simulink model "Task4_Simscape_model"  (R2026a)
settings: Solver=FixedStepAuto  StopTime=8  FixedStep=0.001
model workspace (MATLAB code in the model file):
  | clear; clc; close all;
values from neighbouring files (symbols this model uses):
  A0 = 0.310447780017169    (= 0.310447780017)    [Parameters.m]    (also in Parameters_optimization.m)
  B10 = -0.192075602039053    (= -0.192075602039)    [Parameters.m]    (also in Parameters_optimization.m)
  B20 = -0.011912003704451    (= -0.0119120037045)    [Parameters.m]    (also in Parameters_optimization.m)
  black = partTemplate    [Parameters.m]    (also in Parameters_optimization.m = struct)
  blueBlock = partTemplate    [Parameters.m]    (also in Parameters_optimization.m = struct)
  cyan = partTemplate    [Parameters.m]    (also in Parameters_optimization.m = struct)
  g = 9.81    [Parameters.m]    (also in Parameters_optimization.m)
  G0 = -1.061422531644424    (= -1.06142253164)    [Parameters.m]    (also in Parameters_optimization.m)
  greenBeam = partTemplate    [Parameters.m]    (also in Parameters_optimization.m = struct)
  greenBlock = partTemplate    [Parameters.m]    (also in Parameters_optimization.m = struct)
  grey = partTemplate    [Parameters.m]    (also in Parameters_optimization.m = struct)
  H0 = -0.357470264672538    (= -0.357470264673)    [Parameters.m]    (also in Parameters_optimization.m)
  I0 = -1.033155420835947    (= -1.03315542084)    [Parameters.m]    (also in Parameters_optimization.m)
  JM = 0.002    [Parameters.m]    (also in Parameters_optimization.m)
  LB1 = 0.8    [Parameters.m]    (also in Parameters_optimization.m)
  LB2 = 0.3    [Parameters.m]    (also in Parameters_optimization.m)
  LB3 = 0.24    [Parameters.m]    (also in Parameters_optimization.m)
  Lblack1 = 0.2    [Parameters.m]    (also in Parameters_optimization.m)
  LC1 = 0.4    [Parameters.m]    (also in Parameters_optimization.m)
  LC2 = 0.225    [Parameters.m]    (also in Parameters_optimization.m)
  LG1 = 0.3    [Parameters.m]    (also in Parameters_optimization.m)
  LG2 = 0.8    [Parameters.m]    (also in Parameters_optimization.m)
  Lgrey1 = 1.175    [Parameters.m]    (also in Parameters_optimization.m)
  lightBlue = partTemplate    [Parameters.m]    (also in Parameters_optimization.m = struct)
  LLB1 = 0.248    [Parameters.m]    (also in Parameters_optimization.m)
  LLB2 = 0.235    [Parameters.m]    (also in Parameters_optimization.m)
  LR1 = 1.05    [Parameters.m]    (also in Parameters_optimization.m)
  LW1 = 1.05    [Parameters.m]    (also in Parameters_optimization.m)
  nA = 200    [Parameters.m]    (also in Parameters_optimization.m = 100)
  nB1 = 200    [Parameters.m]    (also in Parameters_optimization.m = 100)
  nB2 = 200    [Parameters.m]    (also in Parameters_optimization.m)
  nG = 20    [Parameters.m]    (also in Parameters_optimization.m)
  nH = 100    [Parameters.m]    (also in Parameters_optimization.m = 50)
  nI = 20    [Parameters.m]    (also in Parameters_optimization.m)
  red = partTemplate    [Parameters.m]    (also in Parameters_optimization.m = struct)
  trajCoeff = coeff    [Parameters.m]    (also in Parameters_optimization.m = [2000 500 1600; Path_Planning_Robot.m)
  trajTime = t    [Parameters.m]    (also in Parameters_optimization.m = [0 2 4 6 8]; Path_Planning_Robot.m)
  w = 0.1    [Parameters.m]    (also in Parameters_optimization.m)
  white = partTemplate    [Parameters.m]    (also in Parameters_optimization.m = struct)
undefined symbols (not defined in the file or in its folder): X, Y, Z
libraries: sm_lib x152, nesl_utility x69, simulink x1
(part 1 of 5)
settings Model: Creator=Bruker  LastModifiedBy=Bruker
settings ExplorerConfigSet: InternalSimMechanicsExplorerSettings=|
  | <ExplorerConfiguration>
  | 
  |   <canonicalview>default</canonicalview>
  | 
  |   <TilePanel>
  |     <TileInfo>
  |       <Tiles Columns="1" Count="1" Height="610" Rows="1" Width="1078">
  |         <Row Weight="1"/>
  |         <Column Weight="1"/>
  |         <Tile Height="1" Width="1" X="0" Y="0"/>
  |       </Tiles>
  |     </TileInfo>
  |     <SceneInfo>
  |       <SceneViewer>
  |         <IsThisViewStd>
  |           <IsStandardView>off</IsStandardView>
  |           <StandardViewName>Front</StandardViewName>
  |         </IsThisViewStd>
  |         <BGColor>
  |           <R>1</R>
  |           <G>1</G>
  |           <B>1</B>
  |           <A>1</A>
  |         </BGColor>
  |         <Camera>
  |           <DoPerspective>off</DoPerspective>
  |           <Position>
  |             <X>0.050962097420724523</X>
  |             <Y>-3.1475704894834529</Y>
  |             <Z>0.37490286963399816</Z>
  |           </Position>
  |           <Center>
  |             <X>0.050962097420724523</X>
  |             <Y>0</Y>
  |             <Z>0.37490286963399816</Z>
  |           </Center>
  |           <Up>
  |             <X>0</X>
  |             <Y>0</Y>
  |             <Z>1</Z>
  |           </Up>
  |           <XLim>0.57510337083613783</XLim>
  |           <YLim>0.57510337083613783</YLim>
  |           <ViewLimDist>0.01</ViewLimDist>
  |         </Camera>
  |       </SceneViewer>
  |     </SceneInfo>
  |   </TilePanel>
  | 
  |   <MechEditorPanel>
  |     <GfxPanelCameraMap/>
  |     <Cameras/>
  |     <VideoCreator>
  |       <IncludeTiles>All</IncludeTiles>
  |       <IncludeTime>on</IncludeTime>
  |       <IncludeWorldFrame>off</IncludeWorldFrame>
  |       <PlaybackSpeedRatio>1</PlaybackSpeedRatio>
  |       <FrameRate>30</FrameRate>
  |       <FrameSize>auto</FrameSize>
  |       <VideoFormat>UncompressedAVI</VideoFormat>
  |     </VideoCreator>
  |   </MechEditorPanel>
  | 
  |   <PlaybackSettings>
  |     <PlaybackSpeedFactor>1</PlaybackSpeedFactor>
  |   </PlaybackSettings>
  | 
  | </ExplorerConfiguration>

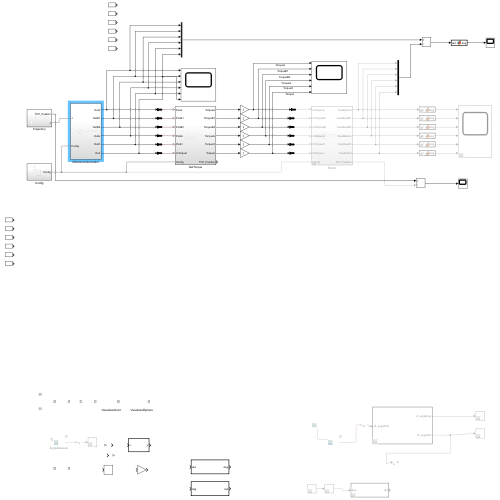
[thumbnail: Simulink's stored preview of the top-level diagram]
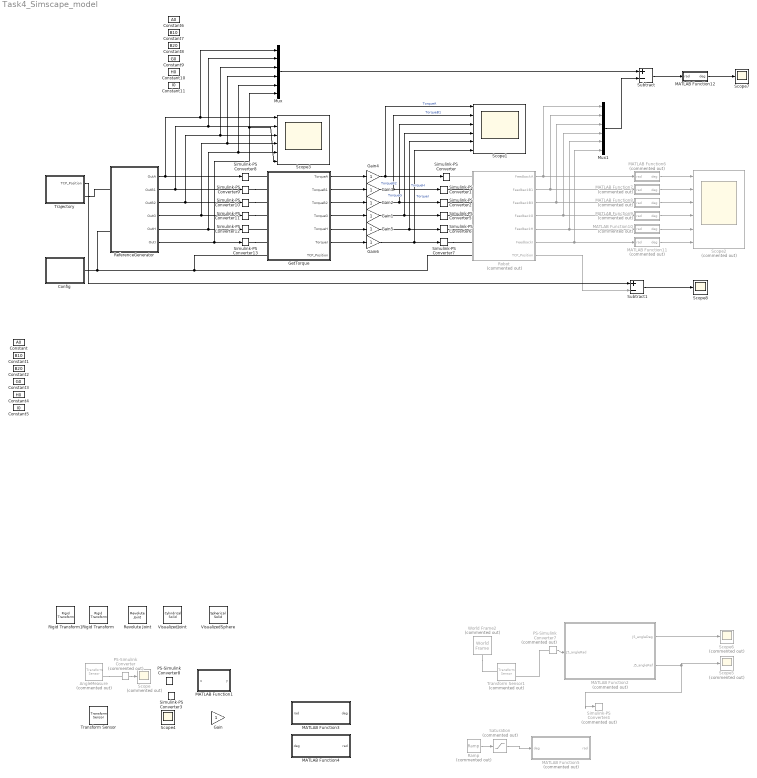
== system Task4_Simscape_model ==
  AngleMeasure : sm_lib/Frames and Transforms/Transform Sensor  Commented=on  MeasurementFrame=World  RotationSequence=XYX  SenseAngle=on  SenseAxis=off  SenseQ=off  SenseR=off  SenseRotationSequence=off  SenseOmegaX=off  SenseOmegaY=off  SenseOmegaZ=off  SenseOmega=off  SenseQDot=off  SenseRDot=off  SenseRotationSequenceDot=off  SenseAlphaX=off  SenseAlphaY=off  SenseAlphaZ=off  SenseAlpha=off  SenseQDDot=off  SenseRDDot=off  SenseX=off  SenseY=off  SenseZ=off  SenseXYZ=off  SenseRad=off  SenseAzim=off  SenseDist=off  SenseInc=off  SenseXDot=off  SenseYDot=off  SenseZDot=off  SenseXYZDot=off  SenseRadDot=off  SenseAzimDot=off  SenseDistDot=off  SenseIncDot=off  SenseXDDot=off  SenseYDDot=off  SenseZDDot=off  SenseXYZDDot=off  SenseRadDDot=off  SenseAzimDDot=off  SenseDistDDot=off  SenseIncDDot=off
  Config : Subsystem
  Constant : Constant  Value=A0
  Constant1 : Constant  Value=B10
  Constant10 : Constant  Value=H0
  Constant11 : Constant  Value=I0
  Constant2 : Constant  Value=B20
  Constant3 : Constant  Value=G0
  Constant4 : Constant  Value=H0
  Constant5 : Constant  Value=I0
  Constant6 : Constant  Value=A0
  Constant7 : Constant  Value=B10
  Constant8 : Constant  Value=B20
  Constant9 : Constant  Value=G0
  Gain{,1..6} (7 alike) : Gain
  GetTorque : Subsystem
  MATLAB Function1 : MATLAB Function  TreatAsAtomicUnit=on
  MATLAB Function10 : MATLAB Function  Commented=on  TreatAsAtomicUnit=on
  MATLAB Function11 : MATLAB Function  Commented=on  TreatAsAtomicUnit=on
  MATLAB Function12 : MATLAB Function  TreatAsAtomicUnit=on
  MATLAB Function2 : MATLAB Function  Commented=on  TreatAsAtomicUnit=on
  MATLAB Function3 : MATLAB Function  TreatAsAtomicUnit=on
  MATLAB Function4 : MATLAB Function  TreatAsAtomicUnit=on
  MATLAB Function5 : MATLAB Function  Commented=on  TreatAsAtomicUnit=on
  MATLAB Function6 : MATLAB Function  Commented=on  TreatAsAtomicUnit=on
  MATLAB Function7 : MATLAB Function  Commented=on  TreatAsAtomicUnit=on
  MATLAB Function8 : MATLAB Function  Commented=on  TreatAsAtomicUnit=on
  MATLAB Function9 : MATLAB Function  Commented=on  TreatAsAtomicUnit=on
  Mux : Mux  Inputs=6
  Mux1 : Mux  Inputs=6
  PS-Simulink Converter : nesl_utility/PS-Simulink Converter  Commented=on  PhysicalDomain=network_engine_domain  SubClassName=ps_output  LeftPortType=input  RightPortType=output  PseudoPeriodic=off  Frequencies=[]  VectorFormat=inherit  Unit=inherit  AffineConversion=off
  PS-Simulink Converter7 : nesl_utility/PS-Simulink Converter  Commented=on  PhysicalDomain=network_engine_domain  SubClassName=ps_output  LeftPortType=input  RightPortType=output  PseudoPeriodic=off  Frequencies=[]  VectorFormat=inherit  Unit=inherit  AffineConversion=off
  PS-Simulink Converter8 : nesl_utility/PS-Simulink Converter  PhysicalDomain=network_engine_domain  SubClassName=ps_output  LeftPortType=input  RightPortType=output  PseudoPeriodic=off  Frequencies=[]  VectorFormat=inherit  Unit=inherit  AffineConversion=off
  Ramp : simulink/Sources/Ramp  Commented=on  slope=1000/8  start=0  InitialOutput=0
  ReferenceGenerator : Subsystem
  Revolute Joint : sm_lib/Joints/Revolute Joint  JointMode=Normal  CompositeWrenchDir=FollowerOnBase  CompositeWrenchFrame=BaseFrame  SenseConstraintForce=off  SenseConstraintTorque=off  SenseTotalForce=off  SenseTotalTorque=off  PositionTargetSpecify=off  PositionTargetPriority=High  PositionTargetValue=0  PositionTargetValueUnits=deg  VelocityTargetSpecify=off  VelocityTargetPriority=High  VelocityTargetValue=0  VelocityTargetValueUnits=deg/s  EquilibriumPosition=0  EquilibriumPositionUnits=deg  SpringStiffness=0  SpringStiffnessUnits=N*m/deg  DampingCoefficient=0  DampingCoefficientUnits=N*m/(deg/s)  LowerLimitSpecify=off  LowerLimitBound=-90  LowerLimitBoundUnits=deg  LowerLimitStiffness=1e4  LowerLimitStiffnessUnits=N*m/deg  LowerLimitDamping=10  LowerLimitDampingUnits=N*m/(deg/s)  LowerLimitTransitionRegionWidth=0.1  LowerLimitTransitionRegionWidthUnits=deg  UpperLimitSpecify=off  UpperLimitBound=90  UpperLimitBoundUnits=deg  UpperLimitStiffness=1e4  UpperLimitStiffnessUnits=N*m/deg  UpperLimitDamping=10  UpperLimitDampingUnits=N*m/(deg/s)  UpperLimitTransitionRegionWidth=0.1  UpperLimitTransitionRegionWidthUnits=deg  TorqueActuationMode=NoTorque  MotionActuationMode=ComputedMotion  SensePosition=off  SenseVelocity=off  SenseAcceleration=off  SenseTorqueForce=off  SenseLowerLimitTorqueForce=off  SenseUpperLimitTorqueForce=off
  Rigid Transform : sm_lib/Frames and Transforms/Rigid Transform  RotationMethod=None  FollAlignAxisA=+X  BaseAlignAxisA=+Y  FollAlignAxisB=+Y  BaseAlignAxisB=+Z  RotationStandardAxis=+Z  RotationAngle=0  RotationAngleUnits=deg  RotationArbitraryAxis=[0 0 1]  RotationSequenceAxes=FollowerAxes  RotationSequence=XYX  RotationSequenceAngles=[0 0 0]  RotationSequenceAnglesUnits=deg  RotationMatrix=[1 0 0;0 1 0;0 0 1]  Quaternion=[1 0 0 0]  TranslationMethod=None  TranslationCartesianOffset=[0 0 0]  TranslationCartesianOffsetUnits=m  TranslationStandardAxis=+Z  TranslationStandardOffset=0  TranslationStandardOffsetUnits=m  TranslationROffset=0  TranslationROffsetUnits=m  TranslationThetaOffset=0  TranslationThetaOffsetUnits=deg  TranslationZOffset=0  TranslationZOffsetUnits=m
  Rigid Transform1 : sm_lib/Frames and Transforms/Rigid Transform  RotationMethod=None  FollAlignAxisA=+X  BaseAlignAxisA=+Y  FollAlignAxisB=+Y  BaseAlignAxisB=+Z  RotationStandardAxis=+Z  RotationAngle=0  RotationAngleUnits=deg  RotationArbitraryAxis=[0 0 1]  RotationSequenceAxes=FollowerAxes  RotationSequence=XYX  RotationSequenceAngles=[0 0 0]  RotationSequenceAnglesUnits=deg  RotationMatrix=[1 0 0;0 1 0;0 0 1]  Quaternion=[1 0 0 0]  TranslationMethod=None  TranslationCartesianOffset=[0 0 0]  TranslationCartesianOffsetUnits=m  TranslationStandardAxis=+Z  TranslationStandardOffset=0  TranslationStandardOffsetUnits=m  TranslationROffset=0  TranslationROffsetUnits=m  TranslationThetaOffset=0  TranslationThetaOffsetUnits=deg  TranslationZOffset=0  TranslationZOffsetUnits=m
  Robot : Subsystem  Commented=on
  Saturation : Saturate  Commented=on  UpperLimit=180  LowerLimit=0
  Scope : Scope  Commented=on
      settings: ActiveDisplayYMinimum=-0.73658474319379863  ActiveDisplayYMaximum=3.1152097370111522
  Scope1 : Scope  NumInputPorts=6
      settings: ActiveDisplayYMinimum=-2952.2267469286785  ActiveDisplayYMaximum=3391.0221732300965  DataLoggingVariableName=ScopeData3
  Scope2 : Scope  Commented=on  NumInputPorts=6
      settings: ActiveDisplayYMinimum=-1272.9618215701389  ActiveDisplayYMaximum=7546.22968605892  DataLoggingVariableName=ScopeData7
  Scope3 : Scope  NumInputPorts=6
      settings: ActiveDisplayYMinimum=-1.8760388198347495  ActiveDisplayYMaximum=1.651358016161629  DataLoggingVariableName=ScopeData8
  Scope4 : Scope
      settings: ActiveDisplayYMinimum=-0.73658474319379863  ActiveDisplayYMaximum=3.1152097370111522  DataLoggingVariableName=ScopeData4
  Scope5 : Scope  Commented=on
      settings: ActiveDisplayYMinimum=-48.192253346240207  ActiveDisplayYMaximum=119.75135174755562  DataLoggingVariableName=ScopeData5
  Scope6 : Scope  Commented=on
      settings: ActiveDisplayYMinimum=31.179110662774175  ActiveDisplayYMaximum=57.893452986332861  DataLoggingVariableName=ScopeData6
  Scope7 : Scope
      settings: ActiveDisplayYMinimum=-0.21970207705285275  ActiveDisplayYMaximum=0.43327861827645181  DataLoggingVariableName=ScopeData9
  Scope8 : Scope
      settings: ActiveDisplayYMinimum=-2.9165642436363033  ActiveDisplayYMaximum=5.0853605029518887  DataLoggingVariableName=ScopeData16
  Simulink-PS Converter{,1..2,5..7} (6 alike) : nesl_utility/Simulink-PS Converter  PhysicalDomain=network_engine_domain  SubClassName=ps_input  LeftPortType=input  RightPortType=output  PseudoPeriodic=off  Frequencies=[]  NoiseDistribution=none  NoiseParameters=[]  Unit=N*m  AffineConversion=off  FilteringAndDerivatives=filter  SimscapeFilterOrder=2  InputFilterTimeConstant=0.001  UdotUserProvided=0
  Simulink-PS Converter{8..13} (6 alike) : nesl_utility/Simulink-PS Converter  PhysicalDomain=network_engine_domain  SubClassName=ps_input  LeftPortType=input  RightPortType=output  PseudoPeriodic=off  Frequencies=[]  NoiseDistribution=none  NoiseParameters=[]  Unit=rad  AffineConversion=off  FilteringAndDerivatives=filter  SimscapeFilterOrder=2  InputFilterTimeConstant=0.001  UdotUserProvided=0
  Simulink-PS Converter3 : nesl_utility/Simulink-PS Converter  PhysicalDomain=network_engine_domain  SubClassName=ps_input  LeftPortType=input  RightPortType=output  PseudoPeriodic=off  Frequencies=[]  NoiseDistribution=none  NoiseParameters=[]  Unit=1  AffineConversion=off  FilteringAndDerivatives=provide  SimscapeFilterOrder=1  InputFilterTimeConstant=0.001  UdotUserProvided=0
  Simulink-PS Converter4 : nesl_utility/Simulink-PS Converter  Commented=on  PhysicalDomain=network_engine_domain  SubClassName=ps_input  LeftPortType=input  RightPortType=output  PseudoPeriodic=off  Frequencies=[]  NoiseDistribution=none  NoiseParameters=[]  Unit=1  AffineConversion=off  FilteringAndDerivatives=filter  SimscapeFilterOrder=2  InputFilterTimeConstant=0.001  UdotUserProvided=0
  Subtract : Sum  Inputs=+-
  Subtract1 : Sum  Inputs=+-
  Trajectory : Subsystem
  Transform Sensor : sm_lib/Frames and Transforms/Transform Sensor  MeasurementFrame=World  RotationSequence=XYX  SenseAngle=off  SenseAxis=off  SenseQ=off  SenseR=off  SenseRotationSequence=off  SenseOmegaX=off  SenseOmegaY=off  SenseOmegaZ=off  SenseOmega=off  SenseQDot=off  SenseRDot=off  SenseRotationSequenceDot=off  SenseAlphaX=off  SenseAlphaY=off  SenseAlphaZ=off  SenseAlpha=off  SenseQDDot=off  SenseRDDot=off  SenseX=off  SenseY=off  SenseZ=off  SenseXYZ=off  SenseRad=off  SenseAzim=off  SenseDist=off  SenseInc=off  SenseXDot=off  SenseYDot=off  SenseZDot=off  SenseXYZDot=off  SenseRadDot=off  SenseAzimDot=off  SenseDistDot=off  SenseIncDot=off  SenseXDDot=off  SenseYDDot=off  SenseZDDot=off  SenseXYZDDot=off  SenseRadDDot=off  SenseAzimDDot=off  SenseDistDDot=off  SenseIncDDot=off
  Transform Sensor1 : sm_lib/Frames and Transforms/Transform Sensor  Commented=on  MeasurementFrame=World  RotationSequence=XYX  SenseAngle=on  SenseAxis=off  SenseQ=off  SenseR=off  SenseRotationSequence=off  SenseOmegaX=off  SenseOmegaY=off  SenseOmegaZ=off  SenseOmega=off  SenseQDot=off  SenseRDot=off  SenseRotationSequenceDot=off  SenseAlphaX=off  SenseAlphaY=off  SenseAlphaZ=off  SenseAlpha=off  SenseQDDot=off  SenseRDDot=off  SenseX=off  SenseY=off  SenseZ=off  SenseXYZ=off  SenseRad=off  SenseAzim=off  SenseDist=off  SenseInc=off  SenseXDot=off  SenseYDot=off  SenseZDot=off  SenseXYZDot=off  SenseRadDot=off  SenseAzimDot=off  SenseDistDot=off  SenseIncDot=off  SenseXDDot=off  SenseYDDot=off  SenseZDDot=off  SenseXYZDDot=off  SenseRadDDot=off  SenseAzimDDot=off  SenseDistDDot=off  SenseIncDDot=off
  VisualizedJoint : sm_lib/Body Elements/Cylindrical Solid  CylinderRadius=w  CylinderRadiusUnits=m  CylinderLength=2*w  CylinderLengthUnits=m  ExportEntireGeometry=off  InertiaType=CalculateFromGeometry  BasedOnType=Density  Density=0  DensityUnits=kg/m^3  Mass=1  MassUnits=kg  CenterOfMass=[0 0 0]  CenterOfMassUnits=m  MomentsOfInertia=[1 1 1]  MomentsOfInertiaUnits=kg*m^2  ProductsOfInertia=[0 0 0]  ProductsOfInertiaUnits=kg*m^2  GraphicType=FromGeometry  MarkerShape=Sphere  MarkerSize=10  GraphicVisPropType=SimpleVisualProperties  GraphicDiffuseColor=[1 0 1]  GraphicOpacity=1  GraphicSpecularColor=[0.5 0.5 0.5 1.0]  GraphicAmbientColor=[0.15 0.15 0.15 1.0]  GraphicEmissiveColor=[0.0 0.0 0.0 1.0]  GraphicShininess=75  DoExposeReferenceFrame=on  SerializedFrames=<Frames/>
  VisualizedSphere : sm_lib/Body Elements/Spherical Solid  SphereRadius=w  SphereRadiusUnits=m  ExportEntireGeometry=off  InertiaType=CalculateFromGeometry  BasedOnType=Density  Density=1000  DensityUnits=kg/m^3  Mass=1  MassUnits=kg  CenterOfMass=[0 0 0]  CenterOfMassUnits=m  MomentsOfInertia=[1 1 1]  MomentsOfInertiaUnits=kg*m^2  ProductsOfInertia=[0 0 0]  ProductsOfInertiaUnits=kg*m^2  GraphicType=FromGeometry  MarkerShape=Sphere  MarkerSize=10  GraphicVisPropType=SimpleVisualProperties  GraphicDiffuseColor=[1 0 1]  GraphicOpacity=1  GraphicSpecularColor=[0.5 0.5 0.5 1.0]  GraphicAmbientColor=[0.15 0.15 0.15 1.0]  GraphicEmissiveColor=[0.0 0.0 0.0 1.0]  GraphicShininess=75  DoExposeReferenceFrame=on  SerializedFrames=<Frames/>
  World Frame2 : sm_lib/Frames and Transforms/World Frame  Commented=on
  wires:
  PS-Simulink Converter/1 -> Scope/1
  PS-Simulink Converter7/1 -> MATLAB Function2/1(J5_angleRad)
  MATLAB Function2/2(J5_angleRef) -> Simulink-PS Converter4/1, Scope5/1
  MATLAB Function2/1(J5_angleDeg) -> Scope6/1
  Ramp/1 -> Saturation/1
  Saturation/1 -> MATLAB Function5/1(deg)
  ReferenceGenerator/1(OutA) -> Simulink-PS Converter8/1, Scope3/1, Mux/1
  ReferenceGenerator/2(OutB1) -> Simulink-PS Converter9/1, Scope3/2, Mux/2
  ReferenceGenerator/4(OutG) -> Simulink-PS Converter11/1, Scope3/4, Mux/4
  ReferenceGenerator/5(OutH) -> Simulink-PS Converter12/1, Scope3/5, Mux/5
  ReferenceGenerator/6(OutI) -> Simulink-PS Converter13/1, Scope3/6, Mux/6
  Robot/1(FeedbackA) -> Mux1/1, MATLAB Function6/1(rad)
  Robot/2(FeedbackB1) -> Mux1/2, MATLAB Function7/1(rad)
  Robot/3(FeedbackB3) -> MATLAB Function8/1(rad), Mux1/3
  Robot/4(FeedbackG) -> MATLAB Function9/1(rad), Mux1/4
  Robot/5(FeedbackH) -> MATLAB Function10/1(rad), Mux1/5
  Robot/6(FeedbackI) -> MATLAB Function11/1(rad), Mux1/6
  ReferenceGenerator/3(OutB2) -> Simulink-PS Converter10/1, Mux/3, Scope3/3
  Subtract/1 -> MATLAB Function12/1(rad)
  Mux/1 -> Subtract/1
  Mux1/1 -> Subtract/2
  Gain1/1 -> Scope1/4, Simulink-PS Converter5/1  "TorqueG"
  Gain2/1 -> Scope1/3, Simulink-PS Converter2/1  "TorqueB2"
  Gain3/1 -> Scope1/2, Simulink-PS Converter1/1  "TorqueB1"
  Gain4/1 -> Simulink-PS Converter/1, Scope1/1  "TorqueA"
  Gain5/1 -> Scope1/5, Simulink-PS Converter6/1  "TorqueH"
  Gain6/1 -> Scope1/6, Simulink-PS Converter7/1  "TorqueI"
  MATLAB Function6/1(deg) -> Scope2/1
  MATLAB Function7/1(deg) -> Scope2/2
  MATLAB Function8/1(deg) -> Scope2/3
  MATLAB Function9/1(deg) -> Scope2/4
  MATLAB Function10/1(deg) -> Scope2/5
  MATLAB Function11/1(deg) -> Scope2/6
  MATLAB Function12/1(deg) -> Scope7/1
  GetTorque/1(TorqueA) -> Gain4/1
  Subtract1/1 -> Scope8/1
  Robot/7(TCP_Position) -> Subtract1/2
  Trajectory/1(TCP_Position) -> Subtract1/1
  GetTorque/2(TorqueB1) -> Gain3/1
  GetTorque/3(TorqueB2) -> Gain2/1
  GetTorque/4(TorqueG) -> Gain1/1
  GetTorque/5(TorqueH) -> Gain5/1
  GetTorque/6(TorqueI) -> Gain6/1
  connections:
  AngleMeasure/RConn2 -- PS-Simulink Converter/LConn1
  World Frame2/RConn1 -- Transform Sensor1/LConn1
  PS-Simulink Converter7/LConn1 -- Transform Sensor1/RConn2
  Trajectory/RConn1 -- ReferenceGenerator/LConn1
  ReferenceGenerator/LConn2 -- Robot/LConn7 -- GetTorque/LConn7 -- Config/RConn1
  Robot/LConn1 -- Simulink-PS Converter/RConn1
  Simulink-PS Converter1/RConn1 -- Robot/LConn2
  Simulink-PS Converter2/RConn1 -- Robot/LConn3
  Simulink-PS Converter5/RConn1 -- Robot/LConn4
  Simulink-PS Converter6/RConn1 -- Robot/LConn5
  Simulink-PS Converter7/RConn1 -- Robot/LConn6
  GetTorque/LConn1 -- Simulink-PS Converter8/RConn1
  Simulink-PS Converter9/RConn1 -- GetTorque/LConn2
  Simulink-PS Converter10/RConn1 -- GetTorque/LConn3
  Simulink-PS Converter11/RConn1 -- GetTorque/LConn4
  GetTorque/LConn5 -- Simulink-PS Converter12/RConn1
  Simulink-PS Converter13/RConn1 -- GetTorque/LConn6

== system Task4_Simscape_model/Config ==
  Mechanism Configuration : sm_lib/Utilities/Mechanism Configuration  UniformGravity=Constant  GravityVector=[0 0 -g]  GravityVectorUnits=m/s^2  LinearizationDelta=0.001  JointModeTransitionNonlinearIterations=2
  Solver Configuration : nesl_utility/Solver Configuration  PhysicalDomain=network_engine_domain  SubClassName=solver  LeftPortType=input  RightPortType=generic  Tones=[]  Harmonics=[]  SimulateNoise=off  Profile=off  UseLocalSampling=off  EnableSwitchedLinearOptims=on  FrequencyDomain=off  UseCCode=off  RelTol=0.001  AbsTol=1e-06  MinStep=1e-09  ToWorkspace=off  RevertToSquareIcSolve=off  NumHomotopyIterations=100  PhasorMode=off  PhasorModeNumHarmonics=1  ConsistencySolver=NEWTON_FTOL  CanonicalOrdering=UNORDERED  OptimizeIntermediates=UNOPTIMIZED  IndexReductionMethod=DerivativeReplacement  DoDC=off  ResidualTolerance=1e-6  ConsistencyTolSource=GLOBAL  ConsistencyAbsTol=0.001  ConsistencyRelTol=0.001  ConsistencyTolFactor=0.001  UseLocalSolver=off  LocalSolverChoice=NE_BACKWARD_EULER_ADVANCER  ResolveIndetEquations=on  FunctionEvalNumThread=1  LocalSolverSampleTime=.001  DoFixedCost=off  MaxNonlinIter=3  MaxModeIter=2  ComputeImpulses=off  ImpulseIterations=2  LinearAlgebra=Sparse  LinearAlgebraNumThread=0  EquationFormulation=NE_TIME_EF  DelaysMemoryBudget=1024  AutomaticFiltering=on  FilteringTimeConstant=0.001  PartitionStorageMethod=AS_NEEDED  PartitionMemoryBudget=1024  PartitionMethod=FAST  MultibodyUseLocalSolver=off  MultibodyLocalSolverChoice=ODE1  MultibodyLocalSolverSampleTime=0.001
  World Frame : sm_lib/Frames and Transforms/World Frame
  Conifg : PMIOPort  Side=Right
  connections:
  Solver Configuration/RConn1 -- Conifg/RConn1 -- Mechanism Configuration/RConn1 -- World Frame/RConn1

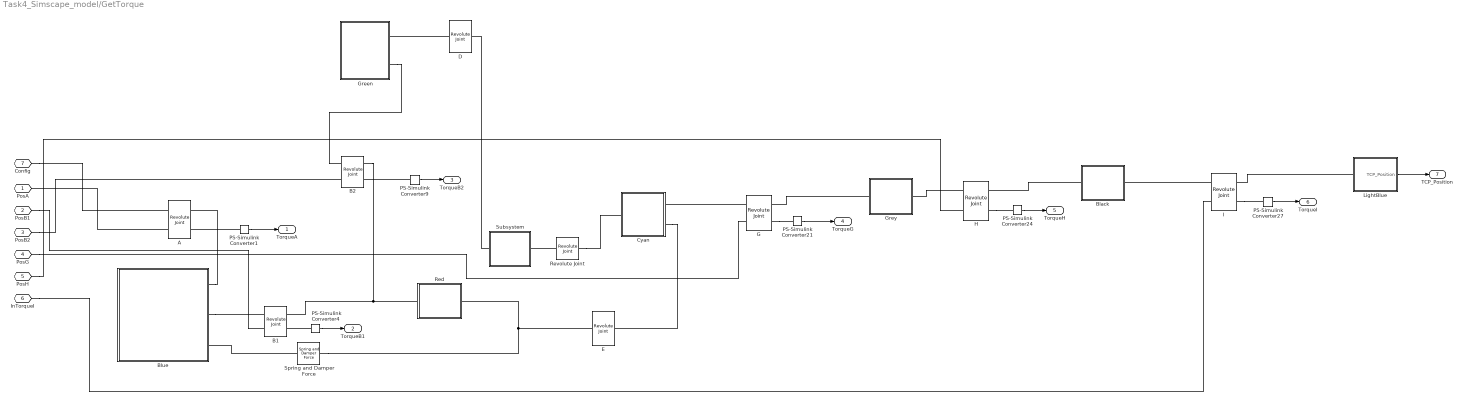
== system Task4_Simscape_model/GetTorque ==
  A : sm_lib/Joints/Revolute Joint  JointMode=Normal  CompositeWrenchDir=FollowerOnBase  CompositeWrenchFrame=BaseFrame  SenseConstraintForce=off  SenseConstraintTorque=off  SenseTotalForce=off  SenseTotalTorque=off  PositionTargetSpecify=off  PositionTargetPriority=High  PositionTargetValue=0  PositionTargetValueUnits=deg  VelocityTargetSpecify=off  VelocityTargetPriority=High  VelocityTargetValue=0  VelocityTargetValueUnits=deg/s  EquilibriumPosition=0  EquilibriumPositionUnits=deg  SpringStiffness=0  SpringStiffnessUnits=N*m/deg  DampingCoefficient=0  DampingCoefficientUnits=N*m/(deg/s)  LowerLimitSpecify=off  LowerLimitBound=-90  LowerLimitBoundUnits=deg  LowerLimitStiffness=1e4  LowerLimitStiffnessUnits=N*m/deg  LowerLimitDamping=10  LowerLimitDampingUnits=N*m/(deg/s)  LowerLimitTransitionRegionWidth=0.1  LowerLimitTransitionRegionWidthUnits=deg  UpperLimitSpecify=off  UpperLimitBound=90  UpperLimitBoundUnits=deg  UpperLimitStiffness=1e4  UpperLimitStiffnessUnits=N*m/deg  UpperLimitDamping=10  UpperLimitDampingUnits=N*m/(deg/s)  UpperLimitTransitionRegionWidth=0.1  UpperLimitTransitionRegionWidthUnits=deg  TorqueActuationMode=ComputedTorque  MotionActuationMode=InputMotion  SensePosition=off  SenseVelocity=off  SenseAcceleration=off  SenseTorqueForce=on  SenseLowerLimitTorqueForce=off  SenseUpperLimitTorqueForce=off
  B1 : sm_lib/Joints/Revolute Joint  JointMode=Normal  CompositeWrenchDir=FollowerOnBase  CompositeWrenchFrame=BaseFrame  SenseConstraintForce=off  SenseConstraintTorque=off  SenseTotalForce=off  SenseTotalTorque=off  PositionTargetSpecify=off  PositionTargetPriority=High  PositionTargetValue=0  PositionTargetValueUnits=deg  VelocityTargetSpecify=off  VelocityTargetPriority=High  VelocityTargetValue=0  VelocityTargetValueUnits=deg/s  EquilibriumPosition=0  EquilibriumPositionUnits=deg  SpringStiffness=0  SpringStiffnessUnits=N*m/deg  DampingCoefficient=0  DampingCoefficientUnits=N*m/(deg/s)  LowerLimitSpecify=on  LowerLimitBound=-80  LowerLimitBoundUnits=deg  LowerLimitStiffness=1e6  LowerLimitStiffnessUnits=N*m/deg  LowerLimitDamping=1000  LowerLimitDampingUnits=N*m/(deg/s)  LowerLimitTransitionRegionWidth=0.1  LowerLimitTransitionRegionWidthUnits=deg  UpperLimitSpecify=on  UpperLimitBound=80  UpperLimitBoundUnits=deg  UpperLimitStiffness=1e6  UpperLimitStiffnessUnits=N*m/deg  UpperLimitDamping=1000  UpperLimitDampingUnits=N*m/(deg/s)  UpperLimitTransitionRegionWidth=0.1  UpperLimitTransitionRegionWidthUnits=deg  TorqueActuationMode=ComputedTorque  MotionActuationMode=InputMotion  SensePosition=off  SenseVelocity=off  SenseAcceleration=off  SenseTorqueForce=on  SenseLowerLimitTorqueForce=off  SenseUpperLimitTorqueForce=off
  B2 : sm_lib/Joints/Revolute Joint  JointMode=Normal  CompositeWrenchDir=FollowerOnBase  CompositeWrenchFrame=BaseFrame  SenseConstraintForce=off  SenseConstraintTorque=off  SenseTotalForce=off  SenseTotalTorque=off  PositionTargetSpecify=off  PositionTargetPriority=High  PositionTargetValue=0  PositionTargetValueUnits=deg  VelocityTargetSpecify=off  VelocityTargetPriority=High  VelocityTargetValue=0  VelocityTargetValueUnits=deg/s  EquilibriumPosition=0  EquilibriumPositionUnits=deg  SpringStiffness=0  SpringStiffnessUnits=N*m/deg  DampingCoefficient=0  DampingCoefficientUnits=N*m/(deg/s)  LowerLimitSpecify=off  LowerLimitBound=-90  LowerLimitBoundUnits=deg  LowerLimitStiffness=1e4  LowerLimitStiffnessUnits=N*m/deg  LowerLimitDamping=10  LowerLimitDampingUnits=N*m/(deg/s)  LowerLimitTransitionRegionWidth=0.1  LowerLimitTransitionRegionWidthUnits=deg  UpperLimitSpecify=off  UpperLimitBound=90  UpperLimitBoundUnits=deg  UpperLimitStiffness=1e4  UpperLimitStiffnessUnits=N*m/deg  UpperLimitDamping=10  UpperLimitDampingUnits=N*m/(deg/s)  UpperLimitTransitionRegionWidth=0.1  UpperLimitTransitionRegionWidthUnits=deg  TorqueActuationMode=ComputedTorque  MotionActuationMode=InputMotion  SensePosition=off  SenseVelocity=off  SenseAcceleration=off  SenseTorqueForce=on  SenseLowerLimitTorqueForce=off  SenseUpperLimitTorqueForce=off
  Black : Subsystem
  Blue : Subsystem
  Cyan : Subsystem
  D : sm_lib/Joints/Revolute Joint  JointMode=Normal  CompositeWrenchDir=FollowerOnBase  CompositeWrenchFrame=BaseFrame  SenseConstraintForce=off  SenseConstraintTorque=off  SenseTotalForce=off  SenseTotalTorque=off  PositionTargetSpecify=off  PositionTargetPriority=High  PositionTargetValue=0  PositionTargetValueUnits=deg  VelocityTargetSpecify=off  VelocityTargetPriority=High  VelocityTargetValue=0  VelocityTargetValueUnits=deg/s  EquilibriumPosition=0  EquilibriumPositionUnits=deg  SpringStiffness=0  SpringStiffnessUnits=N*m/deg  DampingCoefficient=0  DampingCoefficientUnits=N*m/(deg/s)  LowerLimitSpecify=off  LowerLimitBound=-90  LowerLimitBoundUnits=deg  LowerLimitStiffness=1e4  LowerLimitStiffnessUnits=N*m/deg  LowerLimitDamping=10  LowerLimitDampingUnits=N*m/(deg/s)  LowerLimitTransitionRegionWidth=0.1  LowerLimitTransitionRegionWidthUnits=deg  UpperLimitSpecify=off  UpperLimitBound=90  UpperLimitBoundUnits=deg  UpperLimitStiffness=1e4  UpperLimitStiffnessUnits=N*m/deg  UpperLimitDamping=10  UpperLimitDampingUnits=N*m/(deg/s)  UpperLimitTransitionRegionWidth=0.1  UpperLimitTransitionRegionWidthUnits=deg  TorqueActuationMode=NoTorque  MotionActuationMode=ComputedMotion  SensePosition=off  SenseVelocity=off  SenseAcceleration=off  SenseTorqueForce=off  SenseLowerLimitTorqueForce=off  SenseUpperLimitTorqueForce=off
  E : sm_lib/Joints/Revolute Joint  JointMode=Normal  CompositeWrenchDir=FollowerOnBase  CompositeWrenchFrame=BaseFrame  SenseConstraintForce=off  SenseConstraintTorque=off  SenseTotalForce=off  SenseTotalTorque=off  PositionTargetSpecify=off  PositionTargetPriority=High  PositionTargetValue=0  PositionTargetValueUnits=deg  VelocityTargetSpecify=off  VelocityTargetPriority=High  VelocityTargetValue=0  VelocityTargetValueUnits=deg/s  EquilibriumPosition=0  EquilibriumPositionUnits=deg  SpringStiffness=0  SpringStiffnessUnits=N*m/deg  DampingCoefficient=0  DampingCoefficientUnits=N*m/(deg/s)  LowerLimitSpecify=on  LowerLimitBound=-80  LowerLimitBoundUnits=deg  LowerLimitStiffness=1e6  LowerLimitStiffnessUnits=N*m/deg  LowerLimitDamping=100000  LowerLimitDampingUnits=N*m/(deg/s)  LowerLimitTransitionRegionWidth=0.1  LowerLimitTransitionRegionWidthUnits=deg  UpperLimitSpecify=on  UpperLimitBound=80  UpperLimitBoundUnits=deg  UpperLimitStiffness=1e6  UpperLimitStiffnessUnits=N*m/deg  UpperLimitDamping=100000  UpperLimitDampingUnits=N*m/(deg/s)  UpperLimitTransitionRegionWidth=0.1  UpperLimitTransitionRegionWidthUnits=deg  TorqueActuationMode=NoTorque  MotionActuationMode=ComputedMotion  SensePosition=off  SenseVelocity=off  SenseAcceleration=off  SenseTorqueForce=off  SenseLowerLimitTorqueForce=off  SenseUpperLimitTorqueForce=off
  G : sm_lib/Joints/Revolute Joint  JointMode=Normal  CompositeWrenchDir=FollowerOnBase  CompositeWrenchFrame=BaseFrame  SenseConstraintForce=off  SenseConstraintTorque=off  SenseTotalForce=off  SenseTotalTorque=off  PositionTargetSpecify=off  PositionTargetPriority=High  PositionTargetValue=0  PositionTargetValueUnits=deg  VelocityTargetSpecify=off  VelocityTargetPriority=High  VelocityTargetValue=0  VelocityTargetValueUnits=deg/s  EquilibriumPosition=0  EquilibriumPositionUnits=deg  SpringStiffness=0  SpringStiffnessUnits=N*m/deg  DampingCoefficient=0  DampingCoefficientUnits=N*m/(deg/s)  LowerLimitSpecify=off  LowerLimitBound=-90  LowerLimitBoundUnits=deg  LowerLimitStiffness=1e4  LowerLimitStiffnessUnits=N*m/deg  LowerLimitDamping=10  LowerLimitDampingUnits=N*m/(deg/s)  LowerLimitTransitionRegionWidth=0.1  LowerLimitTransitionRegionWidthUnits=deg  UpperLimitSpecify=off  UpperLimitBound=90  UpperLimitBoundUnits=deg  UpperLimitStiffness=1e4  UpperLimitStiffnessUnits=N*m/deg  UpperLimitDamping=10  UpperLimitDampingUnits=N*m/(deg/s)  UpperLimitTransitionRegionWidth=0.1  UpperLimitTransitionRegionWidthUnits=deg  TorqueActuationMode=ComputedTorque  MotionActuationMode=InputMotion  SensePosition=off  SenseVelocity=off  SenseAcceleration=off  SenseTorqueForce=on  SenseLowerLimitTorqueForce=off  SenseUpperLimitTorqueForce=off
  Green : Subsystem
  Grey : Subsystem
  H : sm_lib/Joints/Revolute Joint  JointMode=Normal  CompositeWrenchDir=FollowerOnBase  CompositeWrenchFrame=BaseFrame  SenseConstraintForce=off  SenseConstraintTorque=off  SenseTotalForce=off  SenseTotalTorque=off  PositionTargetSpecify=off  PositionTargetPriority=High  PositionTargetValue=0  PositionTargetValueUnits=deg  VelocityTargetSpecify=off  VelocityTargetPriority=High  VelocityTargetValue=0  VelocityTargetValueUnits=deg/s  EquilibriumPosition=0  EquilibriumPositionUnits=deg  SpringStiffness=0  SpringStiffnessUnits=N*m/deg  DampingCoefficient=0  DampingCoefficientUnits=N*m/(deg/s)  LowerLimitSpecify=on  LowerLimitBound=-90  LowerLimitBoundUnits=deg  LowerLimitStiffness=1e4  LowerLimitStiffnessUnits=N*m/deg  LowerLimitDamping=10  LowerLimitDampingUnits=N*m/(deg/s)  LowerLimitTransitionRegionWidth=0.1  LowerLimitTransitionRegionWidthUnits=deg  UpperLimitSpecify=on  UpperLimitBound=90  UpperLimitBoundUnits=deg  UpperLimitStiffness=1e4  UpperLimitStiffnessUnits=N*m/deg  UpperLimitDamping=10  UpperLimitDampingUnits=N*m/(deg/s)  UpperLimitTransitionRegionWidth=0.1  UpperLimitTransitionRegionWidthUnits=deg  TorqueActuationMode=ComputedTorque  MotionActuationMode=InputMotion  SensePosition=off  SenseVelocity=off  SenseAcceleration=off  SenseTorqueForce=on  SenseLowerLimitTorqueForce=off  SenseUpperLimitTorqueForce=off
  I : sm_lib/Joints/Revolute Joint  JointMode=Normal  CompositeWrenchDir=FollowerOnBase  CompositeWrenchFrame=BaseFrame  SenseConstraintForce=off  SenseConstraintTorque=off  SenseTotalForce=off  SenseTotalTorque=off  PositionTargetSpecify=off  PositionTargetPriority=High  PositionTargetValue=0  PositionTargetValueUnits=deg  VelocityTargetSpecify=off  VelocityTargetPriority=High  VelocityTargetValue=0  VelocityTargetValueUnits=deg/s  EquilibriumPosition=0  EquilibriumPositionUnits=deg  SpringStiffness=0  SpringStiffnessUnits=N*m/deg  DampingCoefficient=0  DampingCoefficientUnits=N*m/(deg/s)  LowerLimitSpecify=off  LowerLimitBound=-90  LowerLimitBoundUnits=deg  LowerLimitStiffness=1e4  LowerLimitStiffnessUnits=N*m/deg  LowerLimitDamping=10  LowerLimitDampingUnits=N*m/(deg/s)  LowerLimitTransitionRegionWidth=0.1  LowerLimitTransitionRegionWidthUnits=deg  UpperLimitSpecify=off  UpperLimitBound=90  UpperLimitBoundUnits=deg  UpperLimitStiffness=1e4  UpperLimitStiffnessUnits=N*m/deg  UpperLimitDamping=10  UpperLimitDampingUnits=N*m/(deg/s)  UpperLimitTransitionRegionWidth=0.1  UpperLimitTransitionRegionWidthUnits=deg  TorqueActuationMode=ComputedTorque  MotionActuationMode=InputMotion  SensePosition=off  SenseVelocity=off  SenseAcceleration=off  SenseTorqueForce=on  SenseLowerLimitTorqueForce=off  SenseUpperLimitTorqueForce=off
  LightBlue : Subsystem
  PS-Simulink Converter{1,4,9,21,24,27} (6 alike) : nesl_utility/PS-Simulink Converter  PhysicalDomain=network_engine_domain  SubClassName=ps_output  LeftPortType=input  RightPortType=output  PseudoPeriodic=off  Frequencies=[]  VectorFormat=inherit  Unit=inherit  AffineConversion=off
  Red : Subsystem
  Revolute Joint : sm_lib/Joints/Revolute Joint  JointMode=Normal  CompositeWrenchDir=FollowerOnBase  CompositeWrenchFrame=BaseFrame  SenseConstraintForce=off  SenseConstraintTorque=off  SenseTotalForce=off  SenseTotalTorque=off  PositionTargetSpecify=off  PositionTargetPriority=High  PositionTargetValue=0  PositionTargetValueUnits=deg  VelocityTargetSpecify=off  VelocityTargetPriority=High  VelocityTargetValue=0  VelocityTargetValueUnits=deg/s  EquilibriumPosition=0  EquilibriumPositionUnits=deg  SpringStiffness=0  SpringStiffnessUnits=N*m/deg  DampingCoefficient=0  DampingCoefficientUnits=N*m/(deg/s)  LowerLimitSpecify=off  LowerLimitBound=-90  LowerLimitBoundUnits=deg  LowerLimitStiffness=1e4  LowerLimitStiffnessUnits=N*m/deg  LowerLimitDamping=10  LowerLimitDampingUnits=N*m/(deg/s)  LowerLimitTransitionRegionWidth=0.1  LowerLimitTransitionRegionWidthUnits=deg  UpperLimitSpecify=off  UpperLimitBound=90  UpperLimitBoundUnits=deg  UpperLimitStiffness=1e4  UpperLimitStiffnessUnits=N*m/deg  UpperLimitDamping=10  UpperLimitDampingUnits=N*m/(deg/s)  UpperLimitTransitionRegionWidth=0.1  UpperLimitTransitionRegionWidthUnits=deg  TorqueActuationMode=NoTorque  MotionActuationMode=ComputedMotion  SensePosition=off  SenseVelocity=off  SenseAcceleration=off  SenseTorqueForce=off  SenseLowerLimitTorqueForce=off  SenseUpperLimitTorqueForce=off
  Spring and Damper Force : sm_lib/Forces and Torques/Spring and Damper Force  NaturalLength=L0_spring  NaturalLengthUnits=m  SpringStiffness=k_spring  SpringStiffnessUnits=N/m  DampingCoefficient=0  DampingCoefficientUnits=N/(m/s)  SenseForce=off
  Subsystem : Subsystem
  PosA : PMIOPort  Side=Left
  PosB1 : PMIOPort  Port=2  Side=Left
  PosB2 : PMIOPort  Port=3  Side=Left
  PosG : PMIOPort  Port=4  Side=Left
  PosH : PMIOPort  Port=5  Side=Left
  InTorqueI : PMIOPort  Port=6  Side=Left
  Config : PMIOPort  Port=7  Side=Left
  TorqueA : Outport
  TorqueB1 : Outport  Port=2
  TorqueB2 : Outport  Port=3
  TorqueG : Outport  Port=4
  TorqueH : Outport  Port=5
  TorqueI : Outport  Port=6
  TCP_Position : Outport  Port=7
  wires:
  LightBlue/1(TCP_Position) -> TCP_Position/1
  PS-Simulink Converter1/1 -> TorqueA/1
  PS-Simulink Converter4/1 -> TorqueB1/1
  PS-Simulink Converter9/1 -> TorqueB2/1
  PS-Simulink Converter21/1 -> TorqueG/1
  PS-Simulink Converter24/1 -> TorqueH/1
  PS-Simulink Converter27/1 -> TorqueI/1
  connections:
  B2/RConn1 -- Red/RConn1 -- B1/RConn1
  LightBlue/LConn1 -- I/RConn1
  G/LConn1 -- Cyan/RConn1
  Spring and Damper Force/RConn1 -- E/LConn1 -- Red/LConn1
  Black/LConn1 -- H/RConn1
  Revolute Joint/LConn1 -- Subsystem/LConn1
  Spring and Damper Force/LConn1 -- Blue/RConn3
  Subsystem/RConn1 -- D/RConn1
  Green/RConn2 -- B2/LConn1
  I/LConn1 -- Black/RConn1
  Blue/RConn2 -- B1/LConn1
  H/LConn1 -- Grey/RConn1
  Revolute Joint/RConn1 -- Cyan/LConn1
  D/LConn1 -- Green/RConn1
  Grey/LConn1 -- G/RConn1
  Blue/RConn1 -- A/RConn1
  Cyan/RConn2 -- E/RConn1
  G/RConn2 -- PS-Simulink Converter21/LConn1
  A/LConn2 -- PosA/RConn1
  PosB1/RConn1 -- B1/LConn2
  PosB2/RConn1 -- B2/LConn2
  PosG/RConn1 -- G/LConn2
  PosH/RConn1 -- H/LConn2
  InTorqueI/RConn1 -- I/LConn2
  Config/RConn1 -- A/LConn1
  PS-Simulink Converter1/LConn1 -- A/RConn2
  PS-Simulink Converter4/LConn1 -- B1/RConn2
  PS-Simulink Converter9/LConn1 -- B2/RConn2
  H/RConn2 -- PS-Simulink Converter24/LConn1
  I/RConn2 -- PS-Simulink Converter27/LConn1
